simulink model "FSI04"  (R2024b)
settings: Solver=ode8  StartTime=0.0  StopTime=t_stop  FixedStep=1e-4  RelTol=1e-3
values from neighbouring files (symbols this model uses):
  b = 350    [FSI03WS.m]    (also in FSI04WS.m = 5; FSI08WS.m = 1.25663706144; FSI09WS.m = 3.14159265359)
  k = 50000    [FSI04WS.m]    (also in FSI08WS.m = 986.960440109; FSI09WS.m = 15791.3670417; FSI10WS.m = 1480)
  m = 70    [FSI03WS.m]    (also in FSI04WS.m = 2; FSI08WS.m = 1; FSI09WS.m = 4; FSI10WS.m = 2)
  omega = omegas(i)    [FSI04WS.m]    (also in FSI05WS.m = out.ScopeData.signals(1).values; FSI06WS.m = out.ScopeData1.signals(1).values; FSI07WS.m = out.ScopeData3.signals(1).values; FSI08WS.m = 31.4159265359)
  switch_con_sin = -1    [FSI04WS.m]
  switch_cs_chirp = -1    [FSI04WS.m]
  t_stop = 500    [FSI04WS.m]    (also in FSI07WS.m = 1; FSI08WS.m = 100; FSI09WS.m = 600; FSI10WS.m = 1)
  x0 = 1    [FSI04WS.m]    (also in FSI08WS.m = 0; FSI09WS.m = 0)
libraries: simulink x2
settings Model: Creator=fmiro  LastModifiedBy=fmiro

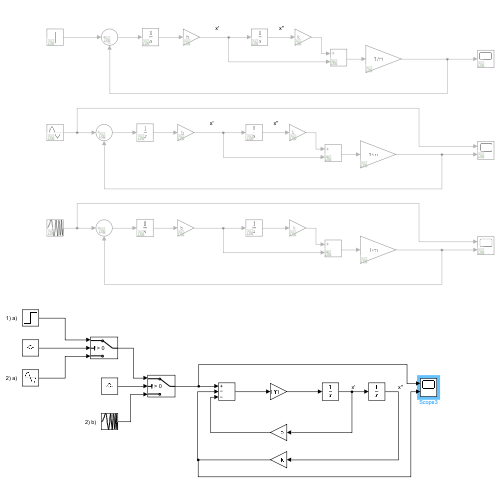
[thumbnail: Simulink's stored preview of the top-level diagram]
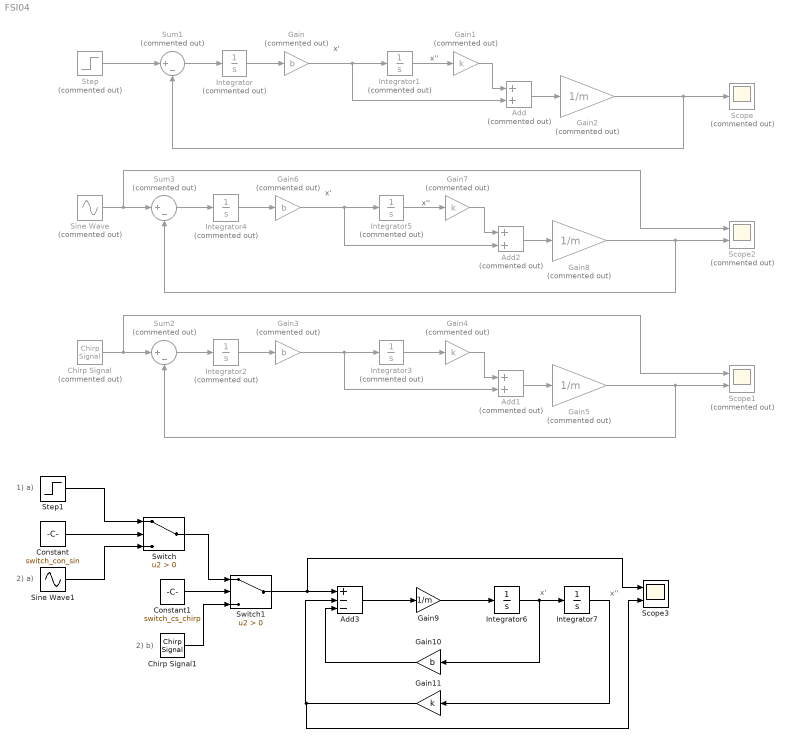
== system FSI04 ==
  note: 2) a)
  note: x''
  note: x'
  note: x'
  note: x''
  note: x''
  note: x'
  note: 1) a)
  note: 2) b)
  Add : Sum  Commented=on
  Add1 : Sum  Commented=on
  Add2 : Sum  Commented=on
  Add3 : Sum  Inputs=+--
  Chirp Signal : simulink/Sources/Chirp Signal  Commented=on  f1=chirp_start  T=3  f2=1
  Chirp Signal1 : simulink/Sources/Chirp Signal  f1=chirp_start  T=t_stop  f2=chirp_end
  Constant : Constant  Value=switch_con_sin
  Constant1 : Constant  Value=switch_cs_chirp
  Gain : Gain  Commented=on  Gain=b
  Gain1 : Gain  Commented=on  Gain=k
  Gain10 : Gain  Gain=b
  Gain11 : Gain  Gain=k
  Gain2 : Gain  Commented=on  Gain=1/m
  Gain3 : Gain  Commented=on  Gain=b
  Gain4 : Gain  Commented=on  Gain=k
  Gain5 : Gain  Commented=on  Gain=1/m
  Gain6 : Gain  Commented=on  Gain=b
  Gain7 : Gain  Commented=on  Gain=k
  Gain8 : Gain  Commented=on  Gain=1/m
  Gain9 : Gain  Gain=1/m
  Integrator{,1..5} (6 alike) : Integrator  Commented=on
  Integrator6 : Integrator
  Integrator7 : Integrator
  Scope : Scope  Commented=on
  Scope1 : Scope  Commented=on  NumInputPorts=2
  Scope2 : Scope  Commented=on  NumInputPorts=2
  Scope3 : Scope  NumInputPorts=2
  Sine Wave : Sin  Commented=on  Frequency=omega  SampleTime=0
  Sine Wave1 : Sin  Frequency=omega  SampleTime=0
  Step : Step  Commented=on  Time=0  After=x0  SampleTime=0
  Step1 : Step  Time=0  After=x0  SampleTime=0
  Sum1 : Sum  Commented=on  Inputs=|+-
  Sum2 : Sum  Commented=on  Inputs=|+-
  Sum3 : Sum  Commented=on  Inputs=|+-
  Switch : Switch  Criteria=u2 > Threshold  SaturateOnIntegerOverflow=off  InputSameDT=off
  Switch1 : Switch  Criteria=u2 > Threshold  SaturateOnIntegerOverflow=off  InputSameDT=off
  wires:
  Add/1 -> Gain2/1
  Gain2/1 -> Scope/1, Sum1/2
  Step/1 -> Sum1/1
  Integrator/1 -> Gain/1
  Sum1/1 -> Integrator/1
  Gain/1 -> Integrator1/1, Add/2
  Integrator1/1 -> Gain1/1
  Gain1/1 -> Add/1
  Gain4/1 -> Add1/1
  Chirp Signal/1 -> Scope1/1, Sum2/1
  Sum2/1 -> Integrator2/1
  Integrator3/1 -> Gain4/1
  Gain3/1 -> Integrator3/1, Add1/2
  Gain5/1 -> Sum2/2, Scope1/2
  Integrator2/1 -> Gain3/1
  Add1/1 -> Gain5/1
  Add2/1 -> Gain8/1
  Sine Wave/1 -> Scope2/1, Sum3/1
  Gain7/1 -> Add2/1
  Gain6/1 -> Integrator5/1, Add2/2
  Integrator4/1 -> Gain6/1
  Integrator5/1 -> Gain7/1
  Gain8/1 -> Sum3/2, Scope2/2
  Sum3/1 -> Integrator4/1
  Step1/1 -> Switch/1
  Sine Wave1/1 -> Switch/3
  Switch/1 -> Switch1/1
  Chirp Signal1/1 -> Switch1/3
  Constant/1 -> Switch/2
  Constant1/1 -> Switch1/2
  Switch1/1 -> Scope3/1, Add3/1
  Add3/1 -> Gain9/1
  Gain9/1 -> Integrator6/1
  Integrator6/1 -> Integrator7/1, Gain10/1
  Gain10/1 -> Add3/3
  Integrator7/1 -> Gain11/1
  Gain11/1 -> Scope3/2, Add3/2
